simulink model "Q4_ObserverTank"  (R2024b)
settings: Solver=FixedStepDiscrete  StartTime=0.0  StopTime=2500  FixedStep=Ts  MaxStep=0.5  RelTol=1e-3
InitFcn:
  | run('tank_design.m')
values from neighbouring files (symbols this model uses):
  A = sys_d.A    [tank_design.m]
  Ab = sysb_d.A    [tank_design.m]
  Bb = sysb_d.B    [tank_design.m]
  Bp = sys_d.B    [tank_design.m]
  Cb = [Cmat 0]    [tank_design.m]
  Cmat = [1 0]    [tank_design.m]
  Dp = [0 0]    [tank_design.m]
  K = Kci(1:2)    [tank_design.m]
  Ki = Kci(3)    [tank_design.m]
  L = place(Ab', Cb', po_d)'    [tank_design.m]
  Ts = 1    [tank_design.m]
undefined symbols (not defined in the file or in its folder): DiscIntNeverNeededParam
settings Model: Creator=mehme  LastModifiedBy=mehme

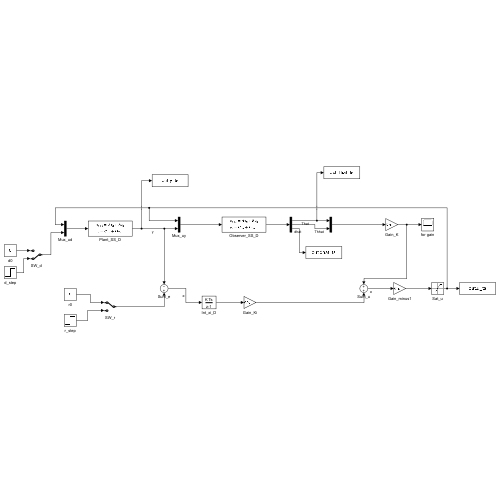
[thumbnail: Simulink's stored preview of the top-level diagram]
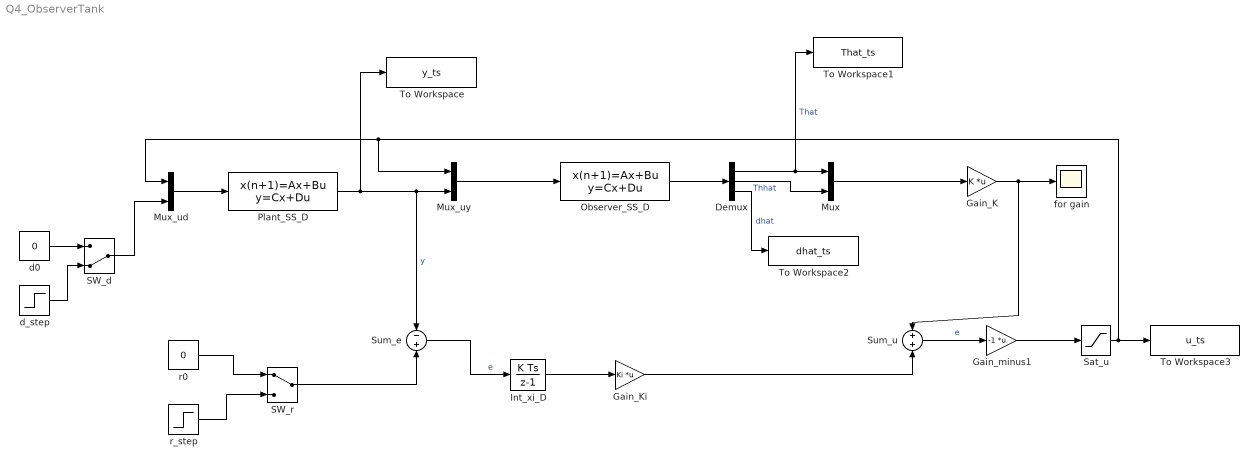
== system Q4_ObserverTank ==
  Demux : Demux  Outputs=3
  Gain_K : Gain  Gain=K  Multiplication=Matrix(K*u)
  Gain_Ki : Gain  Gain=Ki  Multiplication=Matrix(K*u)
  Gain_minus1 : Gain  Gain=-1  Multiplication=Matrix(K*u)
  Int_xi_D : DiscreteIntegrator  SampleTime=Ts  ICPrevOutput=DiscIntNeverNeededParam  ICPrevScaledInput=DiscIntNeverNeededParam
  Mux : Mux  Inputs=2
  Mux_ud : Mux  Inputs=2
  Mux_uy : Mux  Inputs=2
  Observer_SS_D : DiscreteStateSpace  A=Ab - L*Cb  B=[Bb L]  C=eye(3)  D=zeros(3,2)  SampleTime=Ts
  Plant_SS_D : DiscreteStateSpace  A=A  B=Bp  C=Cmat  D=Dp  SampleTime=Ts
  SW_d : ManualSwitch  CurrentSetting=0
  SW_r : ManualSwitch
  Sat_u : Saturate  UpperLimit=15000  LowerLimit=0
  Sum_e : Sum  Inputs=-+
  Sum_u : Sum
  To Workspace : ToWorkspace  VariableName=y_ts  SaveFormat=Timeseries  SampleTime=-1
  To Workspace1 : ToWorkspace  VariableName=That_ts  SaveFormat=Timeseries  SampleTime=-1
  To Workspace2 : ToWorkspace  VariableName=dhat_ts  SaveFormat=Timeseries  SampleTime=-1
  To Workspace3 : ToWorkspace  VariableName=u_ts  SaveFormat=Timeseries  SampleTime=-1
  d0 : Constant  Value=0
  d_step : Step  Time=200  After=800  SampleTime=0
  for gain : Scope
  r0 : Constant  Value=0
  r_step : Step  Time=50  After=10  SampleTime=0
  wires:
  Mux_ud/1 -> Plant_SS_D/1
  SW_d/1 -> Mux_ud/2
  Mux_uy/1 -> Observer_SS_D/1
  Plant_SS_D/1 -> To Workspace/1, Sum_e/1, Mux_uy/2  "y"
  r_step/1 -> SW_r/2
  r0/1 -> SW_r/1
  SW_r/1 -> Sum_e/2
  Sum_e/1 -> Int_xi_D/1  "e"
  Int_xi_D/1 -> Gain_Ki/1
  Gain_K/1 -> for gain/1, Sum_u/1
  Gain_Ki/1 -> Sum_u/2
  Sum_u/1 -> Gain_minus1/1  "e"
  Gain_minus1/1 -> Sat_u/1
  Sat_u/1 -> To Workspace3/1, Mux_uy/1, Mux_ud/1
  Observer_SS_D/1 -> Demux/1
  Demux/1 -> To Workspace1/1, Mux/1  "That"
  Demux/2 -> Mux/2  "Thhat"
  d0/1 -> SW_d/1
  d_step/1 -> SW_d/2
  Mux/1 -> Gain_K/1
  Demux/3 -> To Workspace2/1  "dhat"
